simulink subsystem "Odometry_sub"  (R2023b)
settings: Solver=VariableStepAuto  StartTime=0.0  StopTime=10.0  RelTol=1e-3
undefined symbols (not defined in the file): Motor_Rev_to_Wheel_Distance, Odometry_IC_X, Odometry_IC_Y, Rotation_Local_Inv
libraries: simulink_extras x4, simulink x1
settings Model: Creator=ander  LastModifiedBy=ander

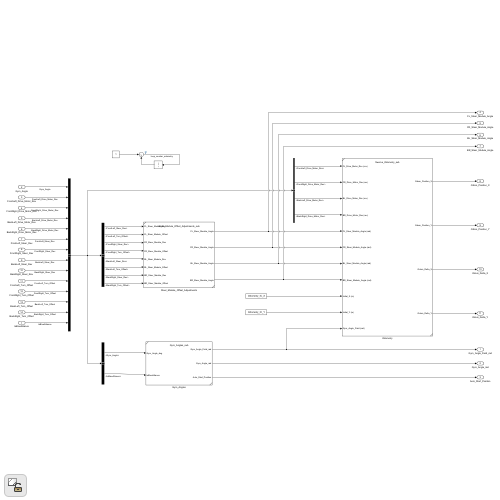
[thumbnail: Simulink's stored preview of the top-level diagram]
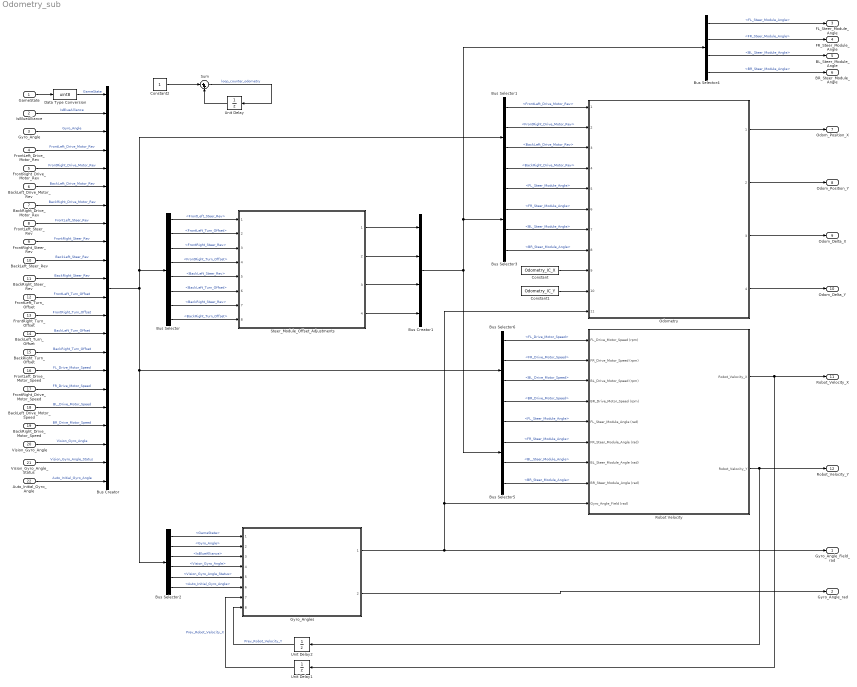
== system Odometry_sub ==
  GameState : Inport
  IsBlueAlliance : Inport  Port=2
  Gyro_Angle : Inport  Port=3
  FrontLeft_Drive_Motor_Rev : Inport  Port=4
  FrontRight_Drive_Motor_Rev : Inport  Port=5
  BackLeft_Drive_Motor_Rev : Inport  Port=6
  BackRight_Drive_Motor_Rev : Inport  Port=7
  FrontLeft_Steer_Rev : Inport  Port=8
  FrontRight_Steer_Rev : Inport  Port=9
  BackLeft_Steer_Rev : Inport  Port=10
  BackRight_Steer_Rev : Inport  Port=11
  FrontLeft_Turn_Offset : Inport  Port=12
  FrontRight_Turn_Offset : Inport  Port=13
  BackLeft_Turn_Offset : Inport  Port=14
  BackRight_Turn_Offset : Inport  Port=15
  FrontLeft_Drive_Motor_Speed : Inport  Port=16
  FrontRight_Drive_Motor_Speed : Inport  Port=17
  BackLeft_Drive_Motor_Speed : Inport  Port=18
  BackRight_Drive_Motor_Speed : Inport  Port=19
  Vision_Gyro_Angle : Inport  Port=20
  Vision_Gyro_Angle_Status : Inport  Port=21
  Auto_Initial_Gyro_Angle : Inport  Port=22
  Bus Creator : BusCreator  Inputs=22
  Bus Creator1 : BusCreator  Inputs=4
  Bus Selector : BusSelector  OutputSignals=FrontLeft_Steer_Rev,FrontLeft_Turn_Offset,FrontRight_Steer_Rev,FrontRight_Turn_Offset,BackLeft_Steer_Rev,BackLeft_Turn_Offset,BackRight_Steer_Rev,BackRight_Turn_Offset
  Bus Selector1 : BusSelector  OutputSignals=FrontLeft_Drive_Motor_Rev,FrontRight_Drive_Motor_Rev,BackLeft_Drive_Motor_Rev,BackRight_Drive_Motor_Rev
  Bus Selector2 : BusSelector  OutputSignals=GameState,Gyro_Angle,IsBlueAlliance,Vision_Gyro_Angle,Vision_Gyro_Angle_Status,Auto_Initial_Gyro_Angle
  Bus Selector3 : BusSelector  OutputSignals=FL_Steer_Module_Angle,FR_Steer_Module_Angle,BL_Steer_Module_Angle,BR_Steer_Module_Angle
  Bus Selector4 : BusSelector  OutputSignals=FL_Steer_Module_Angle,FR_Steer_Module_Angle,BL_Steer_Module_Angle,BR_Steer_Module_Angle
  Bus Selector5 : BusSelector  OutputSignals=FL_Steer_Module_Angle,FR_Steer_Module_Angle,BL_Steer_Module_Angle,BR_Steer_Module_Angle
  Bus Selector6 : BusSelector  OutputSignals=FL_Drive_Motor_Speed,FR_Drive_Motor_Speed,BL_Drive_Motor_Speed,BR_Drive_Motor_Speed
  Constant : Constant  Value=Odometry_IC_X
  Constant1 : Constant  Value=Odometry_IC_Y
  Constant2 : Constant
  Data Type Conversion : DataTypeConversion  OutDataTypeStr=uint8  SaturateOnIntegerOverflow=off  RndMeth=Floor
  Gyro_Angles : Subsystem  ReferencedSubsystem=Gyro_Angles_sub
  Odometry : Subsystem  ReferencedSubsystem=Swerve_Odometry_sub
  Robot Velocity : Subsystem
  Steer_Module_Offset_Adjustments : Subsystem  ReferencedSubsystem=Steer_Module_Offset_Adjustments_sub
  Sum : Sum  Inputs=|++
  Unit Delay : UnitDelay  SampleTime=-1  HasFrameUpgradeWarning=on
  Unit Delay1 : UnitDelay  SampleTime=-1  HasFrameUpgradeWarning=on
  Unit Delay2 : UnitDelay  SampleTime=-1  HasFrameUpgradeWarning=on
  Gyro_Angle_Field_rad : Outport
  Gyro_Angle_rad : Outport  Port=2
  FL_Steer_Module_Angle : Outport  Port=3  OutDataTypeStr=double  Unit=rad
  FR_Steer_Module_Angle : Outport  Port=4  OutDataTypeStr=double  Unit=rad
  BL_Steer_Module_Angle : Outport  Port=5  OutDataTypeStr=double  Unit=rad
  BR_Steer_Module_Angle : Outport  Port=6  OutDataTypeStr=double  Unit=rad
  Odom_Position_X : Outport  Port=7
  Odom_Position_Y : Outport  Port=8
  Odom_Delta_X : Outport  Port=9
  Odom_Delta_Y : Outport  Port=10
  Robot_Velocity_X : Outport  Port=11
  Robot_Velocity_Y : Outport  Port=12
  wires:
  Constant/1 -> Odometry/9
  Constant1/1 -> Odometry/10
  Gyro_Angles/1 -> Gyro_Angle_Field_rad/1, Odometry/11, Robot Velocity/9(Gyro_Angle_Field (rad))
  Odometry/1 -> Odom_Position_X/1
  Odometry/2 -> Odom_Position_Y/1
  Odometry/3 -> Odom_Delta_X/1
  Odometry/4 -> Odom_Delta_Y/1
  Gyro_Angles/2 -> Gyro_Angle_rad/1
  BackRight_Turn_Offset/1 -> Bus Creator/15  "BackRight_Turn_Offset"
  BackLeft_Turn_Offset/1 -> Bus Creator/14  "BackLeft_Turn_Offset"
  FrontRight_Turn_Offset/1 -> Bus Creator/13  "FrontRight_Turn_Offset"
  FrontLeft_Turn_Offset/1 -> Bus Creator/12  "FrontLeft_Turn_Offset"
  BackRight_Steer_Rev/1 -> Bus Creator/11  "BackRight_Steer_Rev"
  BackLeft_Steer_Rev/1 -> Bus Creator/10  "BackLeft_Steer_Rev"
  FrontRight_Steer_Rev/1 -> Bus Creator/9  "FrontRight_Steer_Rev"
  FrontLeft_Steer_Rev/1 -> Bus Creator/8  "FrontLeft_Steer_Rev"
  BackRight_Drive_Motor_Rev/1 -> Bus Creator/7  "BackRight_Drive_Motor_Rev"
  BackLeft_Drive_Motor_Rev/1 -> Bus Creator/6  "BackLeft_Drive_Motor_Rev"
  FrontRight_Drive_Motor_Rev/1 -> Bus Creator/5  "FrontRight_Drive_Motor_Rev"
  FrontLeft_Drive_Motor_Rev/1 -> Bus Creator/4  "FrontLeft_Drive_Motor_Rev"
  Gyro_Angle/1 -> Bus Creator/3  "Gyro_Angle"
  Bus Creator/1 -> Bus Selector2/1, Bus Selector6/1, Bus Selector/1, Bus Selector1/1
  Bus Selector/5 -> Steer_Module_Offset_Adjustments/5  "<BackLeft_Steer_Rev>"
  Bus Selector/4 -> Steer_Module_Offset_Adjustments/4  "<FrontRight_Turn_Offset>"
  Bus Selector/6 -> Steer_Module_Offset_Adjustments/6  "<BackLeft_Turn_Offset>"
  Bus Selector/3 -> Steer_Module_Offset_Adjustments/3  "<FrontRight_Steer_Rev>"
  Bus Selector/7 -> Steer_Module_Offset_Adjustments/7  "<BackRight_Steer_Rev>"
  Bus Selector/2 -> Steer_Module_Offset_Adjustments/2  "<FrontLeft_Turn_Offset>"
  Bus Selector/8 -> Steer_Module_Offset_Adjustments/8  "<BackRight_Turn_Offset>"
  Bus Selector/1 -> Steer_Module_Offset_Adjustments/1  "<FrontLeft_Steer_Rev>"
  Bus Selector1/1 -> Odometry/1  "<FrontLeft_Drive_Motor_Rev>"
  Bus Selector1/2 -> Odometry/2  "<FrontRight_Drive_Motor_Rev>"
  Bus Selector1/3 -> Odometry/3  "<BackLeft_Drive_Motor_Rev>"
  Bus Selector1/4 -> Odometry/4  "<BackRight_Drive_Motor_Rev>"
  Bus Selector2/2 -> Gyro_Angles/2  "<Gyro_Angle>"
  Bus Selector2/3 -> Gyro_Angles/3  "<IsBlueAlliance>"
  Constant2/1 -> Sum/1
  Sum/1 -> Unit Delay/1  "loop_counter_odometry"
  Unit Delay/1 -> Sum/2
  Steer_Module_Offset_Adjustments/4 -> Bus Creator1/4
  Steer_Module_Offset_Adjustments/3 -> Bus Creator1/3
  Steer_Module_Offset_Adjustments/2 -> Bus Creator1/2
  Steer_Module_Offset_Adjustments/1 -> Bus Creator1/1
  Bus Creator1/1 -> Bus Selector3/1, Bus Selector4/1, Bus Selector5/1
  Bus Selector3/4 -> Odometry/8  "<BR_Steer_Module_Angle>"
  Bus Selector3/3 -> Odometry/7  "<BL_Steer_Module_Angle>"
  Bus Selector3/2 -> Odometry/6  "<FR_Steer_Module_Angle>"
  Bus Selector3/1 -> Odometry/5  "<FL_Steer_Module_Angle>"
  Bus Selector4/1 -> FL_Steer_Module_Angle/1  "<FL_Steer_Module_Angle>"
  Bus Selector4/2 -> FR_Steer_Module_Angle/1  "<FR_Steer_Module_Angle>"
  Bus Selector4/3 -> BL_Steer_Module_Angle/1  "<BL_Steer_Module_Angle>"
  Bus Selector4/4 -> BR_Steer_Module_Angle/1  "<BR_Steer_Module_Angle>"
  Bus Selector5/1 -> Robot Velocity/5(FL_Steer_Module_Angle (rad))  "<FL_Steer_Module_Angle>"
  Bus Selector5/2 -> Robot Velocity/6(FR_Steer_Module_Angle (rad))  "<FR_Steer_Module_Angle>"
  Bus Selector5/3 -> Robot Velocity/7(BL_Steer_Module_Angle (rad))  "<BL_Steer_Module_Angle>"
  Bus Selector5/4 -> Robot Velocity/8(BR_Steer_Module_Angle (rad))  "<BR_Steer_Module_Angle>"
  Robot Velocity/1(Robot_Velocity_X) -> Robot_Velocity_X/1, Unit Delay1/1
  Robot Velocity/2(Robot_Velocity_Y) -> Unit Delay2/1, Robot_Velocity_Y/1
  IsBlueAlliance/1 -> Bus Creator/2  "IsBlueAlliance"
  FrontLeft_Drive_Motor_Speed/1 -> Bus Creator/16  "FL_Drive_Motor_Speed"
  FrontRight_Drive_Motor_Speed/1 -> Bus Creator/17  "FR_Drive_Motor_Speed"
  BackLeft_Drive_Motor_Speed/1 -> Bus Creator/18  "BL_Drive_Motor_Speed"
  BackRight_Drive_Motor_Speed/1 -> Bus Creator/19  "BR_Drive_Motor_Speed"
  Bus Selector6/1 -> Robot Velocity/1(FL_Drive_Motor_Speed (rpm))  "<FL_Drive_Motor_Speed>"
  Bus Selector6/2 -> Robot Velocity/2(FR_Drive_Motor_Speed (rpm))  "<FR_Drive_Motor_Speed>"
  Bus Selector6/3 -> Robot Velocity/3(BL_Drive_Motor_Speed (rpm))  "<BL_Drive_Motor_Speed>"
  Bus Selector6/4 -> Robot Velocity/4(BR_Drive_Motor_Speed (rpm))  "<BR_Drive_Motor_Speed>"
  Vision_Gyro_Angle/1 -> Bus Creator/20  "Vision_Gyro_Angle"
  Vision_Gyro_Angle_Status/1 -> Bus Creator/21  "Vision_Gyro_Angle_Status"
  Bus Selector2/4 -> Gyro_Angles/4  "<Vision_Gyro_Angle>"
  Bus Selector2/5 -> Gyro_Angles/5  "<Vision_Gyro_Angle_Status>"
  Unit Delay1/1 -> Gyro_Angles/7  "Prev_Robot_Velocity_X"
  Unit Delay2/1 -> Gyro_Angles/8  "Prev_Robot_Velocity_Y"
  GameState/1 -> Data Type Conversion/1
  Auto_Initial_Gyro_Angle/1 -> Bus Creator/22  "Auto_Initial_Gyro_Angle"
  Data Type Conversion/1 -> Bus Creator/1  "GameState"
  Bus Selector2/6 -> Gyro_Angles/6  "<Auto_Initial_Gyro_Angle>"
  Bus Selector2/1 -> Gyro_Angles/1  "<GameState>"

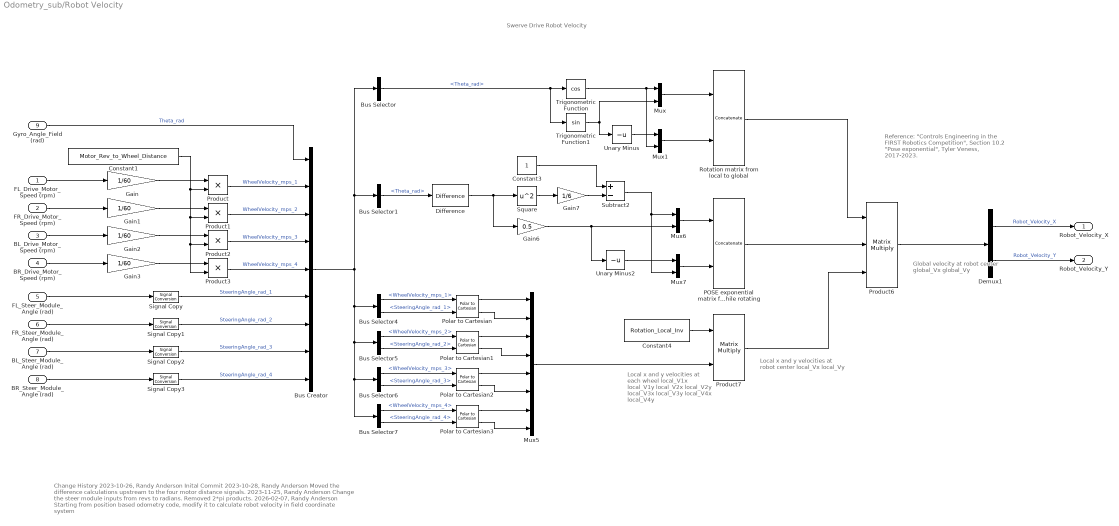
== system Odometry_sub/Robot Velocity ==
  note: Swerve Drive Robot Velocity
  note: Global velocity at
      | robot center
      | global_Vx
      | global_Vy
  note: Reference: "Controls Engineering in the
      |  FIRST Robotics Competition",
      | Section 10.2 "Pose exponential",
      | Tyler Veness, 2017-2023.
  note: Local x and y velocities
      | at robot center
      | local_Vx
      | local_Vy
  note: Change History
      | 2023-10-26, Randy Anderson
      | Inital Commit
      | 2023-10-28, Randy Anderson
      | Moved the difference calculations upstream to the four motor distance signals.
      | 2023-11-25, Randy Anderson
      | Change the steer module inputs from revs to radians. Removed 2*pi products.
      | 2026-02-07, Randy Anderson
      | Starting from position based odometry code, modify it to calculate robot velocity in field coordinate system
  note: Local x and y velocities
      | at each wheel
      | local_V1x
      | local_V1y
      | local_V2x
      | local_V2y
      | local_V3x
      | local_V3y
      | local_V4x
      | local_V4y
  FL_Drive_Motor_Speed (rpm) : Inport
  FR_Drive_Motor_Speed (rpm) : Inport  Port=2
  BL_Drive_Motor_Speed (rpm) : Inport  Port=3
  BR_Drive_Motor_Speed (rpm) : Inport  Port=4
  FL_Steer_Module_Angle (rad) : Inport  Port=5
  FR_Steer_Module_Angle (rad) : Inport  Port=6
  BL_Steer_Module_Angle (rad) : Inport  Port=7
  BR_Steer_Module_Angle (rad) : Inport  Port=8
  Gyro_Angle_Field (rad) : Inport  Port=9
  Bus Creator : BusCreator  Inputs=9
  Bus Selector : BusSelector  OutputSignals=Theta_rad
  Bus Selector1 : BusSelector  OutputSignals=Theta_rad
  Bus Selector4 : BusSelector  OutputSignals=WheelVelocity_mps_1,SteeringAngle_rad_1
  Bus Selector5 : BusSelector  OutputSignals=WheelVelocity_mps_2,SteeringAngle_rad_2
  Bus Selector6 : BusSelector  OutputSignals=WheelVelocity_mps_3,SteeringAngle_rad_3
  Bus Selector7 : BusSelector  OutputSignals=WheelVelocity_mps_4,SteeringAngle_rad_4
  Constant1 : Constant  Value=Motor_Rev_to_Wheel_Distance
  Constant3 : Constant
  Constant4 : Constant  Value=Rotation_Local_Inv
  Demux1 : Demux  Outputs=2
  Difference : simulink/Discrete/Difference  ICPrevInput=0.0  OutMin=[]  OutMax=[]  OutDataType=fixdt(1, 16)  OutScaling=2^-10  DoSatur=off
  Gain{,1..3} (4 alike) : Gain  Gain=1/60
  Gain6 : Gain  Gain=0.5
  Gain7 : Gain  Gain=1/6
  Mux{,1,6..7} (4 alike) : Mux  Inputs=2
  Mux5 : Mux  Inputs=8
  POSE exponential matrix for improved accuracy while rotating : Concatenate  Mode=Multidimensional array  ConcatenateDimension=2
  Polar to Cartesian{,1..3} (4 alike) : simulink_extras/Transformations/Polar to Cartesian
  Product{,1..3} (4 alike) : Product
  Product6 : Product  Inputs=3  Multiplication=Matrix(*)
  Product7 : Product  Multiplication=Matrix(*)
  Rotation matrix from local to global : Concatenate  Mode=Multidimensional array  ConcatenateDimension=2
  Signal Copy{,1..3} (4 alike) : SignalConversion  OverrideOpt=off
  Square : Math  Operator=square
  Subtract2 : Sum  Inputs=+-
  Trigonometric Function : Trigonometry  Operator=cos
  Trigonometric Function1 : Trigonometry
  Unary Minus : UnaryMinus
  Unary Minus2 : UnaryMinus
  Robot_Velocity_X : Outport
  Robot_Velocity_Y : Outport  Port=2
  wires:
  Gain3/1 -> Product3/1
  Gain2/1 -> Product2/1
  Gain1/1 -> Product1/1
  Gain/1 -> Product/1
  Demux1/2 -> Robot_Velocity_Y/1  "Robot_Velocity_Y"
  FR_Drive_Motor_Speed (rpm)/1 -> Gain1/1
  Polar to Cartesian3/2 -> Mux5/8
  Gain6/1 -> Mux6/2, Unary Minus2/1
  Bus Selector6/2 -> Polar to Cartesian2/2  "<SteeringAngle_rad_3>"
  POSE exponential matrix for improved accuracy while rotating/1 -> Product6/2
  Polar to Cartesian1/1 -> Mux5/3
  FL_Drive_Motor_Speed (rpm)/1 -> Gain/1
  Polar to Cartesian/2 -> Mux5/2
  Polar to Cartesian3/1 -> Mux5/7
  Bus Selector6/1 -> Polar to Cartesian2/1  "<WheelVelocity_mps_3>"
  Product1/1 -> Bus Creator/3  "WheelVelocity_mps_2"
  Difference/1 -> Square/1, Gain6/1
  Mux5/1 -> Product7/2
  Square/1 -> Gain7/1
  Mux1/1 -> Rotation matrix from local to global/2
  Mux6/1 -> POSE exponential matrix for improved accuracy while rotating/1
  Mux/1 -> Rotation matrix from local to global/1
  Gain7/1 -> Subtract2/2
  Subtract2/1 -> Mux7/2, Mux6/1
  Bus Selector5/2 -> Polar to Cartesian1/2  "<SteeringAngle_rad_2>"
  Bus Selector1/1 -> Difference/1  "<Theta_rad>"
  Bus Selector4/1 -> Polar to Cartesian/1  "<WheelVelocity_mps_1>"
  Trigonometric Function1/1 -> Unary Minus/1, Mux/2
  Product7/1 -> Product6/3
  BL_Drive_Motor_Speed (rpm)/1 -> Gain2/1
  Unary Minus2/1 -> Mux7/1
  Product3/1 -> Bus Creator/5  "WheelVelocity_mps_4"
  Product6/1 -> Demux1/1
  Unary Minus/1 -> Mux1/1
  Polar to Cartesian/1 -> Mux5/1
  Bus Creator/1 -> Bus Selector/1, Bus Selector1/1, Bus Selector7/1, Bus Selector6/1, Bus Selector5/1, Bus Selector4/1
  Product2/1 -> Bus Creator/4  "WheelVelocity_mps_3"
  Product/1 -> Bus Creator/2  "WheelVelocity_mps_1"
  Rotation matrix from local to global/1 -> Product6/1
  Polar to Cartesian2/2 -> Mux5/6
  Bus Selector5/1 -> Polar to Cartesian1/1  "<WheelVelocity_mps_2>"
  Polar to Cartesian2/1 -> Mux5/5
  Bus Selector7/1 -> Polar to Cartesian3/1  "<WheelVelocity_mps_4>"
  Polar to Cartesian1/2 -> Mux5/4
  FL_Steer_Module_Angle (rad)/1 -> Signal Copy/1
  Constant1/1 -> Product3/2, Product2/2, Product1/2, Product/2
  FR_Steer_Module_Angle (rad)/1 -> Signal Copy1/1
  Mux7/1 -> POSE exponential matrix for improved accuracy while rotating/2
  Bus Selector7/2 -> Polar to Cartesian3/2  "<SteeringAngle_rad_4>"
  Trigonometric Function/1 -> Mux1/2, Mux/1
  Constant4/1 -> Product7/1
  Demux1/1 -> Robot_Velocity_X/1  "Robot_Velocity_X"
  Constant3/1 -> Subtract2/1
  Bus Selector4/2 -> Polar to Cartesian/2  "<SteeringAngle_rad_1>"
  Signal Copy3/1 -> Bus Creator/9  "SteeringAngle_rad_4"
  Bus Selector/1 -> Trigonometric Function1/1, Trigonometric Function/1  "<Theta_rad>"
  Signal Copy1/1 -> Bus Creator/7  "SteeringAngle_rad_2"
  Signal Copy2/1 -> Bus Creator/8  "SteeringAngle_rad_3"
  BR_Drive_Motor_Speed (rpm)/1 -> Gain3/1
  Signal Copy/1 -> Bus Creator/6  "SteeringAngle_rad_1"
  BR_Steer_Module_Angle (rad)/1 -> Signal Copy3/1
  BL_Steer_Module_Angle (rad)/1 -> Signal Copy2/1
  Gyro_Angle_Field (rad)/1 -> Bus Creator/1  "Theta_rad"
